simulink model "furuta_block_model"  (R2026b)
settings: Solver=FixedStepDiscrete  StopTime=5  FixedStep=controlPeriod
model workspace (MAT data in the model file):
  controlPeriod = 0.01
  initialState = [0; 0.174532925199; 0; 0]
  integrationStep = 0.002
  lqrGain = [-0.560244322113 -7.30813603654 -0.304541725168 -0.68699829167]
  maxTorque = 0.03
  plantCoefficients = [0.00019818 0.00016078 0.00016134 0.00013805 0.016934 0.0001 1e-05 0]
  scenarioStimulus = [0 0.0075 0.0175 0.0275 0.0375 0.0475 0.0575 0.0675 0.0775 0.0875 0.0975 0.1075 ... (2004 elements, 501x4)]
  usePolicyCallback = 0
values from neighbouring files (symbols this model uses):
  C = [B A*B A^2*B A^3*B]    [build_furuta_rmd.m]
  N = 20    [build_furuta_rl.m]    (also in design_classical.m)
  pidGains = getVariable(mw,'pidGains')    [check_furuta_lqr_capture.m]
  rmd = struct('model','RMD-X6-P20-60-E','voltage',48,'gearRatio',19.612,          'ratedTorque',20,'ratedCurrent',9.5,'ratedSpeedRPM',153,          'noLoadSpeedRPM',176,'Kt',2.1,'currentLSB',.01)    [build_furuta_rmd.m]
  s = load(matFile,'ds')    [analyze_pi_current_run.m]    (also in analyze_pi_speed_run.m; build_furuta_rl.m = sin(x(2));"; build_furuta_simulink.m = s(1); design_classical.m = furuta_scenarios)
  source = [step '/1']    [add_furuta_plant_blocks.m]    (also in build_furuta_pi.m = get_param(line,'SrcPortHandle'); build_furuta_pi_hardware.m = 'Drive interlocks/3'; compare_furuta_actuators.m = get_param([harness '/Requested torque'],'PortHandles'))
  Z = expm([A B; zeros(1,5)]*p.Ts)    [furuta_linearize.m]
undefined symbols (not defined in the file or in its folder): driveElectrical, lmpcF, lmpcH, poleGain, rlRewardLevel, rmdCommandDelaySamples, sgn, useRmd, X, Y
libraries: sm_lib x36, nesl_utility x8, fl_lib x7, rllib x2, mpclib x1, slpidlib x1, ee_lib x1
(part 1 of 4)
settings Model: Creator=Lsh  LastModifiedBy=Lsh
settings SimscapeCC: SimscapeLogType=all  SimscapeNominalValues="[{\"value\":\"1\",\"unit\":\"A\"},{\"value\":\"1\",\"unit\":\"bar\"},{\"value\":\"1\",\"unit\":\"cm^2\"},{\"value\":\"1\",\"unit\":\"cm^3/s\"},{\"value\":\"1\",\"unit\":\"kJ/kg\"},{\"value\":\"1\",\"unit\":\"kW\"},{\"value\":\"1\",\"unit\":\"l\"},{\"value\":\"1\",\"unit\":\"N\"},{\"value\":\"1\",\"unit\":\"N*m\"},{\"value\":\"1\",\"unit\":\"V\"},{\"value\":\"0.001\",\"unit\":\"Wb\"}]"  SimscapeUseEnergyAccounting=off

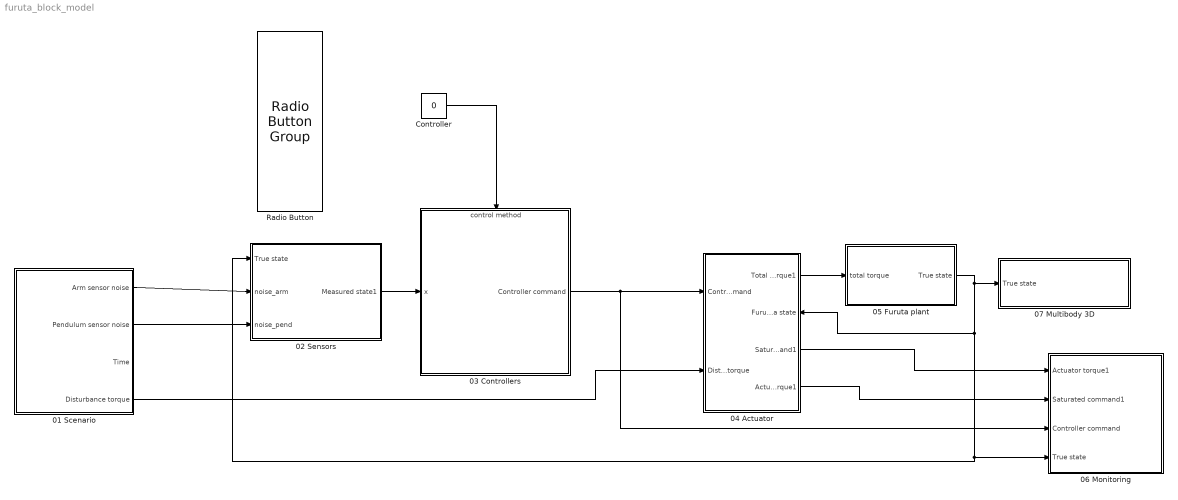
== system furuta_block_model ==
  01 Scenario : Subsystem
  02 Sensors : Subsystem
  03 Controllers : Subsystem
      settings: PortSchema="{\"entries\":[{\"content\":{\"sides\":[{\"content\":{\"connectorIds\":[\"In1\"]},\"type\":\"ConnectorPlacement.EquallySpacedRectSide\",\"uuid\":\"e4b36115-6a1d-4962-9ef8-ed5f31cfcc6a\"},{\"content\":{\"connectorIds\":[\"Out1\"],\"side\":\"RIGHT\"},\"type\":\"ConnectorPlacement.EquallySpacedRectSide\",\"uuid\":\"30852384-c2a0-433b-a443-149c1bfb4c73\"},{\"content\":{\"connectorIds\":[\"In2\"],\"side\":\"TOP\"},\"type\":\"ConnectorPlacement.EquallySpacedRectSide\",\"uuid\":\"d3eba7d3-47d6-4151-b089-0f7eaff5c42c\"},{\"content\":{\"side\":\"BOTTOM\"},\"type\":\"ConnectorPlacement.EquallySpacedRectSide\",\"uuid\":\"8130c781-304c-497e-8c63-b3eca62ccf99\"}]},\"type\":\"ConnectorPlacement.EquallySpacedConnector\",\"uuid\":\"c7c0857b-c1c9-4543-82a8-21998e0f16d7\"}],\"packageUris\":[\"http://schema.mathworks.com/mf0/Connector/R2020b\"],\"version\":\"1.0\"}"
  04 Actuator : Subsystem
      settings: PortSchema="{\"entries\":[{\"content\":{\"sides\":[{\"content\":{\"connectorIds\":[\"In1\",\"In2\"]},\"type\":\"ConnectorPlacement.EquallySpacedRectSide\",\"uuid\":\"22ca9446-42d6-4b29-b122-5af039619f77\"},{\"content\":{\"connectorIds\":[\"Out1\",\"In3\",\"Out2\",\"Out3\"],\"side\":\"RIGHT\"},\"type\":\"ConnectorPlacement.EquallySpacedRectSide\",\"uuid\":\"76c21e35-d24b-4780-9b25-ccc9f5c2777d\"},{\"content\":{\"side\":\"TOP\"},\"type\":\"ConnectorPlacement.EquallySpacedRectSide\",\"uuid\":\"17aac8cc-d921-4d6b-9b67-1213b36be99a\"},{\"content\":{\"side\":\"BOTTOM\"},\"type\":\"ConnectorPlacement.EquallySpacedRectSide\",\"uuid\":\"d916a1b2-62b3-4c8e-90e6-0e905adc1091\"}]},\"type\":\"ConnectorPlacement.EquallySpacedConnector\",\"uuid\":\"4922b9b8-c06b-4aa2-a706-f3caefd4450f\"}],\"packageUris\":[\"http://schema.mathworks.com/mf0/Connector/R2020b\"],\"version\":\"1.0\"}"
  05 Furuta plant : Subsystem
  06 Monitoring : Subsystem
  07 Multibody 3D : Subsystem
  Controller : Constant  Value=0
  Radio Button : RadioButtonGroup  SelectedLabel=PID  ButtonGroupName=Group
  wires:
  01 Scenario/1(Arm sensor noise) -> 02 Sensors/2(noise_arm)
  01 Scenario/2(Pendulum sensor noise) -> 02 Sensors/3(noise_pend)
  03 Controllers/1(Controller command) -> 06 Monitoring/3(Controller command), 04 Actuator/1(Controller command)
  02 Sensors/1(Measured state1) -> 03 Controllers/1(x)
  01 Scenario/4(Disturbance torque) -> 04 Actuator/2(Disturbance torque)
  05 Furuta plant/1(True state) -> 02 Sensors/1(True state), 06 Monitoring/4(True state), 04 Actuator/3(Furuta state), 07 Multibody 3D/1(True state)
  04 Actuator/1(Total torque1) -> 05 Furuta plant/1(total torque)
  04 Actuator/2(Saturated command1) -> 06 Monitoring/1(Actuator torque1)
  04 Actuator/3(Actuator torque1) -> 06 Monitoring/2(Saturated command1)
  Controller/1 -> 03 Controllers/2(control method)

== system furuta_block_model/01 Scenario ==
  Clock : DigitalClock  SampleTime=controlPeriod
  Scenario : FromWorkspace  VariableName=scenarioStimulus  SampleTime=controlPeriod  Interpolate=off  OutputAfterFinalValue=Holding final value
  Scenario channels : Demux  Outputs=3
  Arm sensor noise : Outport
  Pendulum sensor noise : Outport  Port=2
  Time : Outport  Port=3
  Disturbance torque : Outport  Port=4
  wires:
  Scenario channels/1 -> Arm sensor noise/1  "Arm sensor noise"
  Clock/1 -> Time/1  "Time"
  Scenario/1 -> Scenario channels/1
  Scenario channels/3 -> Disturbance torque/1  "Disturbance torque"
  Scenario channels/2 -> Pendulum sensor noise/1  "Pendulum sensor noise"

== system furuta_block_model/02 Sensors ==
  True state : Inport
  noise_arm : Inport  Port=2
  noise_pend : Inport  Port=3
  Measured pendulum : Sum
  Measured pendulum1 : Sum
  Measured state : Mux
  State channels : Demux
  Measured state1 : Outport
  wires:
  True state/1 -> State channels/1
  State channels/1 -> Measured pendulum1/1  "Arm angle"
  Measured state/1 -> Measured state1/1  "Measured state"
  State channels/2 -> Measured pendulum/1  "Pendulum angle"
  Measured pendulum1/1 -> Measured state/1
  Measured pendulum/1 -> Measured state/2
  State channels/4 -> Measured state/4
  State channels/3 -> Measured state/3
  noise_arm/1 -> Measured pendulum1/2
  noise_pend/1 -> Measured pendulum/2

== system furuta_block_model/03 Controllers ==
  x : Inport
  control method : Inport  Port=2
  Controller bank : MultiPortSwitch  DataPortOrder=Zero-based contiguous  Inputs=5  zeroidx=on  SaturateOnIntegerOverflow=off  InputSameDT=off
  LMPC (sim) : Subsystem  Commented=on
  LQR : Subsystem
  MPC Controller : Subsystem
  PID : Subsystem
  PPO : Subsystem
  Pendulum and arm PD : Subsystem  Commented=on
  Pole placement : Subsystem  Commented=on
  SAC : Subsystem
  Controller command : Outport
  wires:
  PPO/1(Out1) -> Controller bank/5
  control method/1 -> PID/1(mode), SAC/2(mode), PPO/1(x), LQR/1(mode), Controller bank/1
  LQR/1(u) -> Controller bank/3
  Controller bank/1 -> Controller command/1
  PID/1(u) -> Controller bank/2
  MPC Controller/1(mv) -> Controller bank/4
  x/1 -> SAC/1(x), PPO/2(mode), PID/2(x), LQR/2(x), MPC Controller/1(mo or x)
  SAC/1(Out1) -> Controller bank/6

== system furuta_block_model/04 Actuator ==
  note: Parameters
      | RMD-X6-P20-60-E
      |
      | Gear Ratio
      | 19.612
      |
      | Input Voltage (V)
      | 48
      |
      | No Load Speed (RPM)
      | 176
      |
      | No Load Input Current (A)
      | 0.9
      |
      | Rated Speed (RPM)
      | 153
      |
      | Rated Torque (N·m)
      | 20
      |
      | Rated Output Power (W)
      | 320
      |
      | Rated Phase Current
      | 9.5
      |
      | (A rms)
      |
      | Peak Torque (N·m)
      | 60
      |
      | Peak Phase Current
      | 29.1
      |
      | (A rms)
      |
      | Efficiency (%)
      | 72.7
      |
      | Motor Back-EMF Constant (Vdc/Krpm)
      | 16
      |
      | Module Torque Constant (N·m/A)
      | 2.1
      |
      | Motor Phase Resistance (Ω)
      | 0.41
      |
      | Motor Phase Inductance (mH)
      | 0.51
      |
      | Pole Pair
      | 10
      |
      | 3 Phase Connection
      | Y
      |
      | Back Drive Torque (N·m)
      | 1.6
      |
      | Backlash (Arcmin)
      | 10
      |
      | Output Bearing Type
      | Crossed Roller Bearings
      |
      | Axial Load - Tension (kN)
      | 1.8
      |
      | Axial Load - Compression (kN)
      | 0.8
      |
      | Radial Load (kN)
      | 2
      |
      | Inertia (Kg·cm²)
      | 0.66
      |
      | Dual Encoder Type & Interface
      | ABS-17BIT (Input) / 17BIT (Output)
      |
      | Repeat Position Accuracy (°)
      | < 0.01
      |
      | Communication
      | EtherCAT
      |
      | Weight (kg)
      | 0.82
      |
      | Insulation Grade
      | F
  Controller command : Inport
  Disturbance torque : Inport  Port=2
  Furuta state : Inport  Port=3
  Actuator limits1 : Saturate  UpperLimit=1  LowerLimit=-1
  Add disturbance1 : Sum
  Applied torque log : ToWorkspace  VariableName=appliedTorqueTrace  SampleTime=-1
  Extract arm speed : Fcn  Expr=u(3)
  RMD X6 P20 60 E : Subsystem
  Select actuator : Switch  Threshold=0.5  SaturateOnIntegerOverflow=off  InputSameDT=off
  Torque Nm1 : Gain  Gain=maxTorque
  Use RMD : Constant  Value=useRmd
  Total torque1 : Outport
  Saturated command1 : Outport  Port=2
  Actuator torque1 : Outport  Port=3
  wires:
  Disturbance torque/1 -> Add disturbance1/2
  Torque Nm1/1 -> Select actuator/3, RMD X6 P20 60 E/2(Requested torque)  "Actuator torque"
  Furuta state/1 -> Extract arm speed/1
  Use RMD/1 -> Select actuator/2
  Controller command/1 -> Actuator limits1/1
  Extract arm speed/1 -> RMD X6 P20 60 E/1(Output shaft speed)
  Actuator limits1/1 -> Torque Nm1/1, Saturated command1/1  "Saturated command"
  RMD X6 P20 60 E/1(Output torque) -> Select actuator/1
  Select actuator/1 -> Actuator torque1/1, Add disturbance1/1, Applied torque log/1
  Add disturbance1/1 -> Total torque1/1  "Total torque"

== system furuta_block_model/05 Furuta plant ==
  total torque : Inport
  Plant state : UnitDelay  InitialCondition=initialState  SampleTime=controlPeriod
  RK4 Furuta plant : Subsystem
  True state : Outport
  wires:
  RK4 Furuta plant/1(next state) -> Plant state/1
  Plant state/1 -> True state/1, RK4 Furuta plant/1(state)  "True state"
  total torque/1 -> RK4 Furuta plant/2(total torque)

== system furuta_block_model/06 Monitoring ==
  Actuator torque1 : Inport
  Saturated command1 : Inport  Port=2
  Controller command : Inport  Port=3
  True state : Inport  Port=4
  Action log : ToWorkspace  VariableName=actionTrace  SampleTime=-1
  Angle signals : Mux  Inputs=2
  Arm and pendulum : Scope
  Arm deg : Gain  Gain=180/pi
  Command log : ToWorkspace  VariableName=commandTrace  SampleTime=-1
  Control torque : Scope
  Pendulum deg : Fcn  Expr=atan2(sin(u),cos(u))*180/pi
  State channels : Demux
  State log : ToWorkspace  VariableName=stateTrace  SampleTime=-1
  Unused rates : Terminator
  Unused rates1 : Terminator
  wires:
  Controller command/1 -> Command log/1
  True state/1 -> State log/1, State channels/1
  Saturated command1/1 -> Control torque/1
  Actuator torque1/1 -> Action log/1
  Angle signals/1 -> Arm and pendulum/1
  Pendulum deg/1 -> Angle signals/2
  Arm deg/1 -> Angle signals/1
  State channels/1 -> Arm deg/1  "Arm angle"
  State channels/2 -> Pendulum deg/1  "Pendulum angle"
  State channels/4 -> Unused rates/1
  State channels/3 -> Unused rates1/1
